simulink subsystem "PickingObj"  (R2026a)
settings: Solver=VariableStepAuto
libraries: nesl_utility x2, sm_lib x1
settings Model: Creator=Dell  LastModifiedBy=Carlos Fabian
settings SimscapeCC: SimscapeNominalValues="[{\"value\":\"1\",\"unit\":\"A\"},{\"value\":\"1\",\"unit\":\"bar\"},{\"value\":\"1\",\"unit\":\"cm^2\"},{\"value\":\"1\",\"unit\":\"cm^3/s\"},{\"value\":\"1\",\"unit\":\"kJ/kg\"},{\"value\":\"1\",\"unit\":\"kW\"},{\"value\":\"1\",\"unit\":\"l\"},{\"value\":\"1\",\"unit\":\"N\"},{\"value\":\"1\",\"unit\":\"N*m\"},{\"value\":\"1\",\"unit\":\"V\"}]"  SimscapeLogType=none  SimscapeLogDataHistory=5000.0

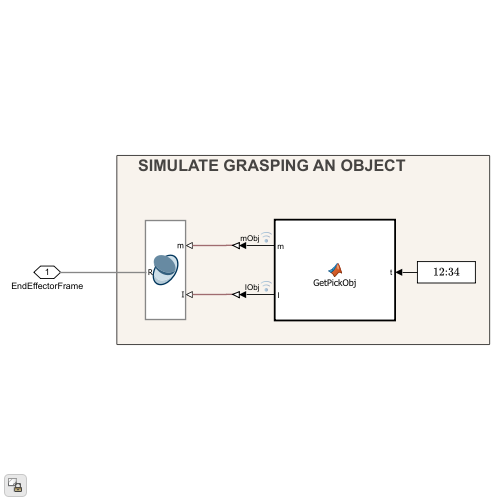
[thumbnail: Simulink's stored preview of the top-level diagram]
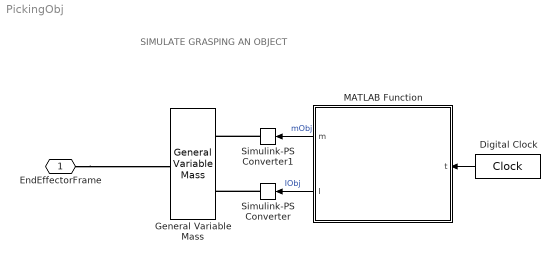
== system PickingObj ==
  note: SIMULATE GRASPING AN OBJECT
  Digital Clock : DigitalClock  SampleTime=0.01
  General Variable Mass : sm_lib/Body Elements/Variable Mass/General Variable Mass  VariableInertiaType=Custom  MassType=TimeVarying  Mass=1  MassUnits=kg  CenterOfMassType=Constant  CenterOfMass=[0 0 0]  CenterOfMassUnits=m  InertiaMatrixType=TimeVarying  MomentsOfInertia=[1 1 1]  MomentsOfInertiaUnits=kg*m^2  ProductsOfInertia=[0 0 0]  ProductsOfInertiaUnits=kg*m^2  GraphicType=InertiaEllipsoid  MarkerShape=Sphere  MarkerSize=10  GraphicVisPropType=SimpleVisualProperties  GraphicDiffuseColor=[1 0 0]  GraphicOpacity=1.0  GraphicSpecularColor=[0.5 0.5 0.5 1.0]  GraphicAmbientColor=[0.15 0.15 0.15 1.0]  GraphicEmissiveColor=[0.0 0.0 0.0 1.0]  GraphicShininess=75
  MATLAB Function : MATLAB Function  TreatAsAtomicUnit=on
  Simulink-PS Converter : nesl_utility/Simulink-PS Converter  PhysicalDomain=network_engine_domain  SubClassName=ps_input  LeftPortType=input  RightPortType=output  PseudoPeriodic=off  Frequencies=[]  NoiseDistribution=none  NoiseParameters=[]  Unit=1  AffineConversion=off  FilteringAndDerivatives=provide  SimscapeFilterOrder=1  InputFilterTimeConstant=0.001  UdotUserProvided=0
  Simulink-PS Converter1 : nesl_utility/Simulink-PS Converter  PhysicalDomain=network_engine_domain  SubClassName=ps_input  LeftPortType=input  RightPortType=output  PseudoPeriodic=off  Frequencies=[]  NoiseDistribution=none  NoiseParameters=[]  Unit=1  AffineConversion=off  FilteringAndDerivatives=provide  SimscapeFilterOrder=1  InputFilterTimeConstant=0.001  UdotUserProvided=0
  EndEffectorFrame : PMIOPort  Side=Left
  wires:
  MATLAB Function/2(I) -> Simulink-PS Converter/1  "IObj"
  MATLAB Function/1(m) -> Simulink-PS Converter1/1  "mObj"
  Digital Clock/1 -> MATLAB Function/1(t)
  connections:
  EndEffectorFrame/RConn1 -- General Variable Mass/RConn1
  Simulink-PS Converter/RConn1 -- General Variable Mass/LConn2
  Simulink-PS Converter1/RConn1 -- General Variable Mass/LConn1

== matlab function PickingObj/MATLAB Function ==
  data: t input; PickObj parameter; m output; I output
function [m,I] = GetPickObj(t, PickObj)

Times = PickObj.Time;

if length(Times) == 2
    cond = t <= Times(1) || t >= Times(2);
else
    cond = t <= Times(1);
end

if ~cond
    m = PickObj.Mass;
    r = PickObj.Radius;
    I1 = 2/5*m*r^2;
    I = diag([I1, I1, I1]);
else
    m = 0;
    I = zeros(3, 3);
end

end
